simulink model "chaine_filtree_sim"  (R2023b)
settings: Solver=FixedStepDiscrete  StartTime=0.0  StopTime=Nbq*L/2  FixedStep=1  RelTol=1e-3
undefined symbols (not defined in the file): hcoef, L, sigq2
libraries: dspsigops x1
settings Model: Creator=e2507457  LastModifiedBy=e2507457

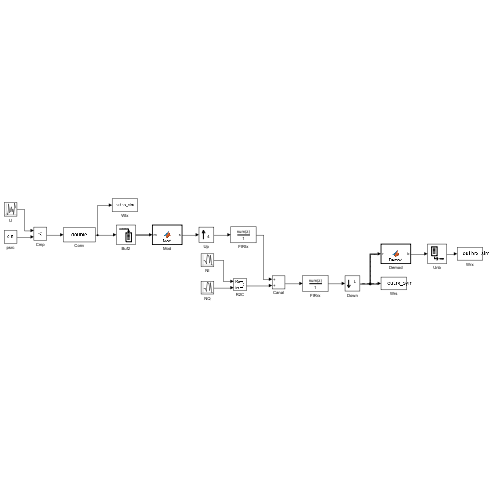
[thumbnail: Simulink's stored preview of the top-level diagram]
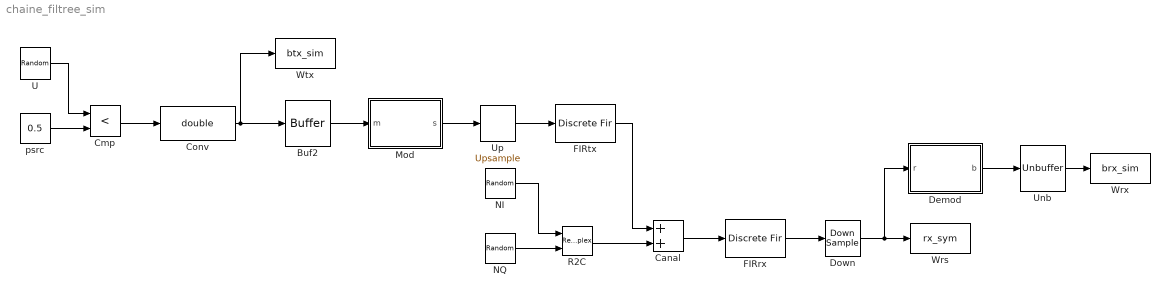
== system chaine_filtree_sim ==
  Buf2 : Buffer  N=2
  Canal : Sum
  Cmp : RelationalOperator  Operator=<  OutDataTypeStr=boolean  RndMeth=Simplest  InputSameDT=off
  Conv : DataTypeConversion  OutDataTypeStr=double  SaturateOnIntegerOverflow=off  RndMeth=Floor
  Demod : MATLAB Function  TreatAsAtomicUnit=on
  Down : DownSample  N=L  phase=phs  AllowArbitraryFixedInput=on
  FIRrx : DiscreteFir  Coefficients=hcoef
  FIRtx : DiscreteFir  Coefficients=hcoef
  Mod : MATLAB Function  TreatAsAtomicUnit=on
  NI : RandomNumber  Variance=sigq2  Seed=22  SampleTime=1
  NQ : RandomNumber  Variance=sigq2  Seed=23  SampleTime=1
  R2C : RealImagToComplex
  U : UniformRandomNumber  Minimum=0  Seed=21  SampleTime=L/2
  Unb : Unbuffer
  Up : dspsigops/Upsample  FactorSource=Dialog parameter  N=L  Nmax=16  phase=0  InputProcessing=Columns as channels (frame based)  RateOptions=Enforce single-rate processing  ic=0  mode=Unused parameter value
  Wrs : ToWorkspace  VariableName=rx_sym  SampleTime=-1
  Wrx : ToWorkspace  VariableName=brx_sim  SampleTime=-1
  Wtx : ToWorkspace  VariableName=btx_sim  SampleTime=-1
  psrc : Constant  Value=0.5  SampleTime=L/2
  wires:
  U/1 -> Cmp/1
  psrc/1 -> Cmp/2
  Cmp/1 -> Conv/1
  Mod/1(s) -> Up/1
  Conv/1 -> Buf2/1, Wtx/1
  Buf2/1 -> Mod/1(m)
  Down/1 -> Wrs/1, Demod/1(r)
  Up/1 -> FIRtx/1
  NQ/1 -> R2C/2
  NI/1 -> R2C/1
  FIRtx/1 -> Canal/1
  R2C/1 -> Canal/2
  Canal/1 -> FIRrx/1
  FIRrx/1 -> Down/1
  Demod/1(b) -> Unb/1
  Unb/1 -> Wrx/1

== matlab function chaine_filtree_sim/Mod ==
  data: m input; s output
function s = Mod(m)
%#codegen
s = complex((1-2*m(1))/sqrt(2), (1-2*m(2))/sqrt(2));
end

== matlab function chaine_filtree_sim/Demod ==
  data: r input; b output
function b = Demod(r)
%#codegen
b = [double(real(r) < 0); double(imag(r) < 0)];
end
